simulink model "sanxiangbanbozhengliudianlu_R"  (R2025a)
settings: Solver=ode23tb  StartTime=0.0  StopTime=0.5  MaxStep=1e-5  RelTol=1e-5
libraries: spsMultimeterLib x4, spsACVoltageSourceLib x3, spsThyristorLib x3, spsMeanLib x1, spsSeriesRLCBranchLib x1, spspowerguiLib x1
settings Model: Creator=小鱼  LastModifiedBy=小鱼

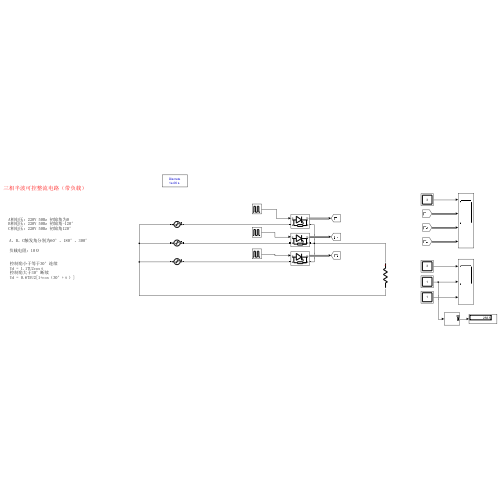
[thumbnail: Simulink's stored preview of the top-level diagram]
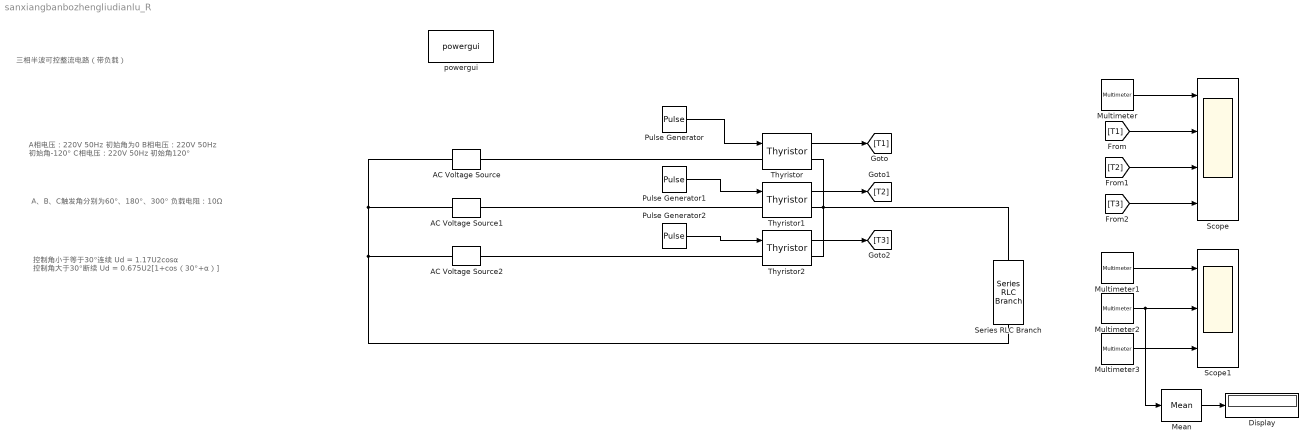
== system sanxiangbanbozhengliudianlu_R ==
  note: 控制角小于等于30°连续
      | Ud = 1.17U2cosα
      | 控制角大于30°断续
      | Ud = 0.675U2[1+cos（30°+α）]
  note: A、B、C触发角分别为60°、180°、300°
      |
      | 负载电阻：10Ω
  note: A相电压：220V 50Hz 初始角为0
      | B相电压：220V 50Hz 初始角-120°
      | C相电压：220V 50Hz 初始角120°
  note: 三相半波可控整流电路（带负载）
  AC Voltage Source : spsACVoltageSourceLib/AC Voltage Source  Amplitude=220*sqrt(2)  Phase=0  Frequency=50  SampleTime=-1  Measurements=Voltage  BusType=swing  Pref=10e3  Qref=0  Qmin=-inf  Qmax=+inf
  AC Voltage Source1 : spsACVoltageSourceLib/AC Voltage Source  Amplitude=220*sqrt(2)  Phase=-120  Frequency=50  SampleTime=-1  Measurements=Voltage  BusType=swing  Pref=10e3  Qref=0  Qmin=-inf  Qmax=+inf
  AC Voltage Source2 : spsACVoltageSourceLib/AC Voltage Source  Amplitude=220*sqrt(2)  Phase=120  Frequency=50  SampleTime=-1  Measurements=Voltage  BusType=swing  Pref=10e3  Qref=0  Qmin=-inf  Qmax=+inf
  Display : Display
  Mean : spsMeanLib/Mean  Freq=150  Vinit=0  Ts=0
  Multimeter : spsMultimeterLib/Multimeter  L=5  sel=[2 3 4]  yselected={}  Gain=[1 1 1]  OutputType=Complex  PlotAtSimulationStop=off  PhasorSimulation=off
  Multimeter1 : spsMultimeterLib/Multimeter  L=5  sel=[2 3 4]  yselected={}  Gain=[1 1 1]  OutputType=Complex  PlotAtSimulationStop=off  PhasorSimulation=off
  Multimeter2 : spsMultimeterLib/Multimeter  L=5  sel=1  yselected={}  Gain=1  OutputType=Complex  PlotAtSimulationStop=off  PhasorSimulation=off
  Multimeter3 : spsMultimeterLib/Multimeter  L=5  sel=5  yselected={}  Gain=1  OutputType=Complex  PlotAtSimulationStop=off  PhasorSimulation=off
  Pulse Generator : DiscretePulseGenerator  PulseType=Time based  Period=0.02  PulseWidth=5  PhaseDelay=30/360*0.02
  Pulse Generator1 : DiscretePulseGenerator  PulseType=Time based  Period=0.02  PulseWidth=5  PhaseDelay=(30+120)/360*0.02
  Pulse Generator2 : DiscretePulseGenerator  PulseType=Time based  Period=0.02  PulseWidth=5  PhaseDelay=(30+240)/360*0.02
  Scope : Scope  NumInputPorts=4
      settings: ActiveDisplayYMinimum=-341.04435778194642  ActiveDisplayYMaximum=384.9136384119609
  Scope1 : Scope  NumInputPorts=3
      settings: ActiveDisplayYMinimum=-344.56316338958771  ActiveDisplayYMaximum=381.39483280431938
  Series RLC Branch : spsSeriesRLCBranchLib/Series RLC Branch  LConnTagsString=__new0  RConnTagsString=__new0  BranchType=R  Resistance=10  Inductance=1e-3  SetiL0=off  InitialCurrent=0  Capacitance=1e-6  Setx0=off  InitialVoltage=0  Measurements=Branch voltage and current
  Thyristor : spsThyristorLib/Thyristor  Ron=0.001  Lon=0  Vf=0.8  IC=0  Rs=500  Cs=250e-9  Measurements=on
  Thyristor1 : spsThyristorLib/Thyristor  Ron=0.001  Lon=0  Vf=0.8  IC=0  Rs=500  Cs=250e-9  Measurements=on
  Thyristor2 : spsThyristorLib/Thyristor  Ron=0.001  Lon=0  Vf=0.8  IC=0  Rs=500  Cs=250e-9  Measurements=on
  powergui : spspowerguiLib/powergui  Priority=1  SimulationMode=Discrete  SampleTime=1e-6  frequency=60  Iterations=50  frequencyindice=50  Pbase=100e6  ErrMax=1e-4  UnitsV=kV  UnitsW=MW  buscounter=0  FunctionMessages=off  echomessages=off  EnableUseOfTLC=off  CurrentSourceSwitches=off  DisableSnubberDevices=off  DisableRonSwitches=off  DisableVfSwitches=off  DisplayEquations=off  AutomaticDiscreteSolvers=off  SolverType=Tustin/Backward Euler (TBE)  Interpol=off  ExternalGateDelay=off  methode=off  Ts=100  x0status=blocks  SPID=on  SwTol=0  HookPort=off  NonlinearTolerance=1e-4  nMaxIteration=100  ContinueOnMaxIteration=off  RestoreLinks=warning  ResistiveCurrentMeasurement=off  Frange=[0:2:500]  Ylog=off  Xlog=on  ShowGrid=off  save=off  variable=ZData  structure=0  ZoomFFT=off  StartTime=0.0  cycles=1  DisplayStyle=1  fundamental=60  FreqAxis=off  MaxFrequency=1000  frequencyindicesteady=1  RmsSteady=1  display=off
  wires:
  Pulse Generator/1 -> Thyristor/1
  Pulse Generator1/1 -> Thyristor1/1
  Pulse Generator2/1 -> Thyristor2/1
  Thyristor/1 -> [T1]
  Thyristor1/1 -> [T2]
  Thyristor2/1 -> [T3]
  [T2] -> Scope/3
  [T1] -> Scope/2
  [T3] -> Scope/4
  Multimeter/1 -> Scope/1
  Multimeter2/1 -> Mean/1, Scope1/2
  Multimeter1/1 -> Scope1/1
  Multimeter3/1 -> Scope1/3
  Mean/1 -> Display/1
  connections:
  AC Voltage Source/RConn1 -- Thyristor/LConn1
  AC Voltage Source1/RConn1 -- Thyristor1/LConn1
  AC Voltage Source2/RConn1 -- Thyristor2/LConn1
  AC Voltage Source/LConn1 -- Series RLC Branch/RConn1 -- AC Voltage Source2/LConn1 -- AC Voltage Source1/LConn1
  Thyristor/RConn1 -- Thyristor2/RConn1 -- Series RLC Branch/LConn1 -- Thyristor1/RConn1
